simulink model "water_level_plant"  (R2023b)
settings: Solver=ode45  StartTime=0.0  StopTime=Tend  MaxStep=0.05  RelTol=1e-6
model workspace (MAT data in the model file):
  A = 0.0576
  H = 0.26
  Ki = 0
  Kp = 20
  Lmax = 80
  Lmin = 30
  Qc = 2.5e-05
  Qmax = 0.000416666666667
  Qol = 0.000416666666667
  SP = 50
  Tend = 900
  Ts = 0.1
  dead = 0.2
  delay = 1.5
  drain = 1
  h0 = 0.026
  kout = 0.000133588971814
  modeSel = 1
  outGravity = 1
  resPct = 1.15384615385
  tDrain = 400
  tauP = 0.3
libraries: slpidlib x1
settings Model: Creator=odyssix  LastModifiedBy=odyssix
settings ModelReferenceCC: UpdateModelReferenceTargets=IfOutOfDate
settings RTWCC: GPUComputeCapability=5.0
settings ConfigComp: CovBoundaryAbsTol=1.0e-5

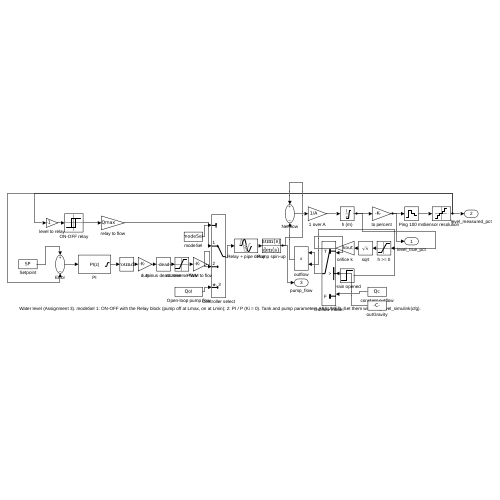
[thumbnail: Simulink's stored preview of the top-level diagram]
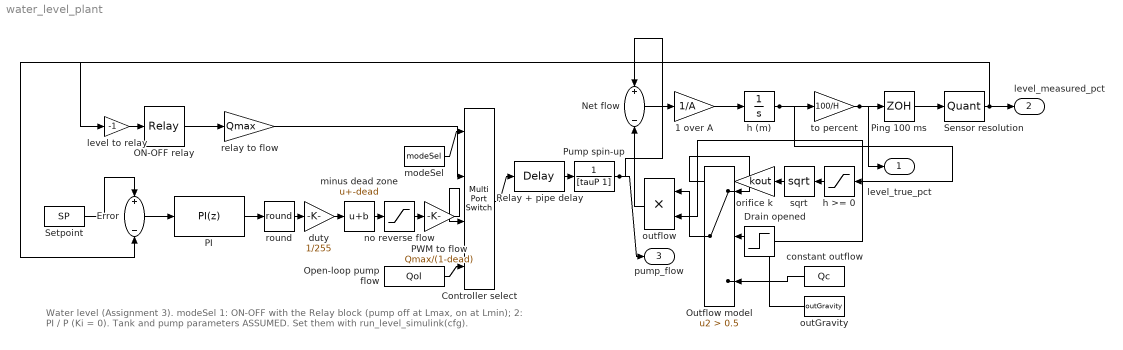
== system water_level_plant ==
  note: Water level (Assignment 3). modeSel 1: ON-OFF with the Relay block (pump off at Lmax, on at Lmin); 2: PI / P (Ki = 0). Tank and pump parameters ASSUMED. Set them with run_level_simulink(cfg).
  1 over A : Gain  Gain=1/A
  Controller select : MultiPortSwitch  SaturateOnIntegerOverflow=off  InputSameDT=off
  Drain opened : Step  Time=tDrain  Before=1  After=drain  SampleTime=0
  Error : Sum  Inputs=+-
  Net flow : Sum  Inputs=+-
  ON-OFF relay : Relay  OnSwitchValue=-Lmin+1e-9  OffSwitchValue=-Lmax-1e-9
  Open-loop pump flow : Constant  Value=Qol
  Outflow model : Switch  Criteria=u2 > Threshold  Threshold=0.5  SaturateOnIntegerOverflow=off  InputSameDT=off
  PI : slpidlib/PID Controller  Controller=PI  Form=Parallel  TimeDomain=Discrete-time  UseExternalTs=off  SampleTime=Ts  IntegratorMethod=Backward Euler  FilterMethod=Forward Euler  ControllerParametersSource=internal  P=Kp  I=Ki  UseKiTs=off  D=0  N=100  UseFilter=on  TunerSelectOption=Transfer Function Based (PID Tuner App)  InitialConditionSource=internal  InitialConditionForIntegrator=0  InitialConditionForFilter=0  DifferentiatorICPrevScaledInput=0  ExternalReset=none  TrackingMode=off  Kt=1  LimitOutput=on  SatLimitsSource=internal  UpperSaturationLimit=255  LowerSaturationLimit=0  LinearizeAsGain=off  AntiWindupMode=clamping  Kb=1  LimitIntegrator=off  UpperIntegratorSaturationLimit=inf  LowerIntegratorSaturationLimit=-inf  POutMin=[]  POutMax=[]  IOutMin=[]  IOutMax=[]  DOutMin=[]  DOutMax=[]  NOutMin=[]  NOutMax=[]  SumOutMin=[]  SumOutMax=[]  SaturationOutMin=[]  SaturationOutMax=[]  PParamMin=[]  PParamMax=[]  IParamMin=[]  IParamMax=[]  DParamMin=[]  DParamMax=[]  NParamMin=[]  NParamMax=[]  KbParamMin=[]  KbParamMax=[]  KtParamMin=[]  KtParamMax=[]  KbOutMin=[]  KbOutMax=[]  KtOutMin=[]  KtOutMax=[]  IntegratorOutMin=[]  IntegratorOutMax=[]  FilterOutMin=[]  FilterOutMax=[]  SumI1OutMin=[]  SumI1OutMax=[]  SumI2OutMin=[]  SumI2OutMax=[]  SumI3OutMin=[]  SumI3OutMax=[]  SumI4OutMin=[]  SumI4OutMax=[]  SumDOutMin=[]  SumDOutMax=[]  DifferentiatorOutMin=[]  DifferentiatorOutMax=[]  FilterDiffOutCoefMin=[]  FilterDiffOutCoefMax=[]  ReciprocalOutMin=[]  ReciprocalOutMax=[]  SumDenOutMin=[]  SumDenOutMax=[]  SumNumOutMin=[]  SumNumOutMax=[]  DivideOutMin=[]  DivideOutMax=[]  UdiffTsProdOutMin=[]  UdiffTsProdOutMax=[]  NTsProdOutMin=[]  NTsProdOutMax=[]  UintegralTsProdOutMin=[]  UintegralTsProdOutMax=[]  UngainTsProdOutMin=[]  UngainTsProdOutMax=[]  ClampingZeroOutDataTypeStr=Inherit: Inherit via back propagation  ClampingZeroOutMin=[]  ClampingZeroOutMax=[]  FilterDenConstantOutDataTypeStr=Inherit: Inherit via back propagation  FilterDenConstantOutMin=[]  FilterDenConstantOutMax=[]  PCopyOutDataTypeStr=Inherit: Inherit via back propagation  PCopyOutMin=[]  PCopyOutMax=[]  NCopyOutDataTypeStr=Inherit: Inherit via back propagation  NCopyOutMin=[]  NCopyOutMax=[]  IntegratorContinuousStateAttributes=''  IntegratorStateMustResolveToSignalObject=off  IntegratorRTWStateStorageClass=Auto  FilterContinuousStateAttributes=''  FilterStateMustResolveToSignalObject=off  FilterRTWStateStorageClass=Auto  ParallelPVariant=InternalParameters  IdealPVariant=Disabled  IVariant=InternalParameters  DVariant=Disabled  IntegratorVariant=Discrete  SatVariant=Enabled  AWVariant=DiscClampingParallel  PCopyVariant=Disabled  TRVariant=Disabled  FdbkBlocksVariant=Feedback  IdealPFdbkVariant=Passthrough  SatFdbkVariant=Passthrough  DerivativeFilterVariant=Disabled  NVariant=Disabled  NCopyVariant=Disabled_SignalSpec  FilterICVariant=Disabled  IntegratorICVariant=InternalICs  ExternalResetVariant=Disabled  TRSumVariant=Passthrough  SumFdbkVariant=Enabled  SumVariant=Sum_PI  TsampFilterVariant=InternalTs  TsampNgainVariant=Passthrough  TsampIntegralVariant=Disabled_SignalSpec  ExternalSaturationOutDataTypeStr=Inherit: Same as second input
      settings: LibrarySourceBlock=simulink/Discrete/Discrete PID Controller
  PWM to flow : Gain  Gain=Qmax/(1-dead)
  Ping 100 ms : ZeroOrderHold  SampleTime=Ts
  Pump spin-up : TransferFcn  Denominator=[tauP 1]
  Relay + pipe delay : TransportDelay  DelayTime=delay  BufferSize=4096
  Sensor resolution : Quantizer  QuantizationInterval=resPct
  Setpoint : Constant  Value=SP
  constant outflow : Constant  Value=Qc
  duty : Gain  Gain=1/255
  h (m) : Integrator  InitialCondition=h0  LimitOutput=on  UpperSaturationLimit=H  LowerSaturationLimit=0
  h >= 0 : Saturate  UpperLimit=inf  LowerLimit=0
  level to relay : Gain  Gain=-1
  minus dead zone : Bias  Bias=-dead  SaturateOnIntegerOverflow=off
  modeSel : Constant  Value=modeSel
  no reverse flow : Saturate  UpperLimit=inf  LowerLimit=0
  orifice k : Gain  Gain=kout
  outGravity : Constant  Value=outGravity
  outflow : Product
  relay to flow : Gain  Gain=Qmax
  round : Rounding  Operator=round
  sqrt : Math  Operator=sqrt
  to percent : Gain  Gain=100/H
  level_true_pct : Outport
  level_measured_pct : Outport  Port=2
  pump_flow : Outport  Port=3
  wires:
  Net flow/1 -> 1 over A/1
  1 over A/1 -> h (m)/1
  h (m)/1 -> h >= 0/1, to percent/1
  h >= 0/1 -> sqrt/1
  sqrt/1 -> orifice k/1
  orifice k/1 -> Outflow model/1
  outGravity/1 -> Outflow model/2
  constant outflow/1 -> Outflow model/3
  Outflow model/1 -> outflow/1
  Drain opened/1 -> outflow/2
  outflow/1 -> Net flow/2
  to percent/1 -> Ping 100 ms/1, level_true_pct/1
  Ping 100 ms/1 -> Sensor resolution/1
  Sensor resolution/1 -> level_measured_pct/1, level to relay/1, Error/2
  level to relay/1 -> ON-OFF relay/1
  ON-OFF relay/1 -> relay to flow/1
  Setpoint/1 -> Error/1
  Error/1 -> PI/1
  PI/1 -> round/1
  round/1 -> duty/1
  duty/1 -> minus dead zone/1
  minus dead zone/1 -> no reverse flow/1
  no reverse flow/1 -> PWM to flow/1
  modeSel/1 -> Controller select/1
  relay to flow/1 -> Controller select/2
  PWM to flow/1 -> Controller select/3
  Open-loop pump flow/1 -> Controller select/4
  Controller select/1 -> Relay + pipe delay/1
  Relay + pipe delay/1 -> Pump spin-up/1
  Pump spin-up/1 -> Net flow/1, pump_flow/1
